simulink model "orig_exp_pid"  (R2023a)
settings: Solver=ode4  StartTime=0.0  StopTime=10  FixedStep=0.0001  RelTol=1e-3
settings Model: Creator=Anonymous  LastModifiedBy=Anonymous

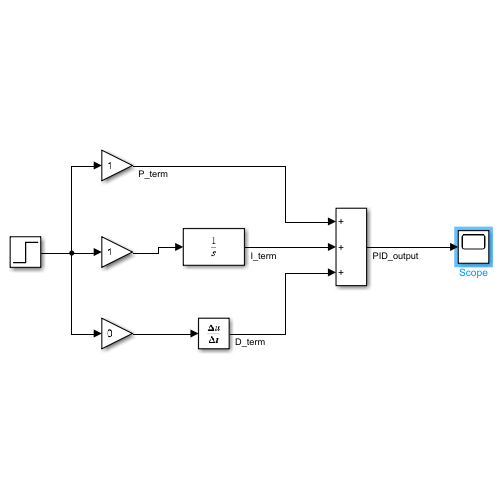
[thumbnail: Simulink's stored preview of the top-level diagram]
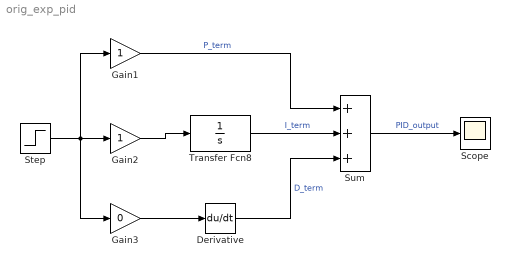
== system orig_exp_pid ==
  Derivative : Derivative
  Gain1 : Gain
  Gain2 : Gain
  Gain3 : Gain  Gain=0
  Scope : Scope
  Step : Step  SampleTime=0
  Sum : Sum  Inputs=+++
  Transfer Fcn8 : TransferFcn  Numerator=1  Denominator=[1 0]
  wires:
  Sum/1 -> Scope/1  "PID_output"
  Derivative/1 -> Sum/3  "D_term"
  Gain3/1 -> Derivative/1
  Transfer Fcn8/1 -> Sum/2  "I_term"
  Gain2/1 -> Transfer Fcn8/1
  Gain1/1 -> Sum/1  "P_term"
  Step/1 -> Gain3/1, Gain2/1, Gain1/1
